simulink model "tg9"  (R2022a)
settings: Solver=ode15s  StartTime=0.0  StopTime=10  MaxStep=0.01  RelTol=1e-3
InitFcn:
  | mecha_param2
  | control_param0
values from neighbouring files (symbols this model uses):
  b0 = 0    [sim_IMMC.m]
  b1 = 1    [sim_IMMC.m]
  back0 = 0    [sim_IMMC.m]
  back1 = 0    [sim_IMMC.m]
  boff = 0    [sim_IMMC.m]
  bon = 0    [sim_IMMC.m]
  c = 0.05    [mecha_param2.m]
  c_jointstop = 0.3 / (pi/180)    (= 17.1887338539)    [mecha_param2.m]
  calctalus = sqrt((L_foot - (DJ1x_foot))^2 + (H_foot-r_cs)^2)    [mecha_param2.m]
  calctoes = sqrt((H_foot-r_cs)^2 + (DJ1x_foot)^2)    [mecha_param2.m]
  corrD = 0.001    [control_param0.m]
  DG_HAT = 0.35    [mecha_param2.m]
  DG_thigh = 0.28    [mecha_param2.m]
  DJ1x_foot = 0.16-r_cs    (= 0.135)    [mecha_param2.m]
  eref = 0.04    [mecha_param2.m]
  FmaxBFSH = 350    [mecha_param2.m]
  FmaxGAS = 1500    [mecha_param2.m]
  FmaxGLU = 1500    [mecha_param2.m]
  FmaxHAM = 3000    [mecha_param2.m]
  FmaxHFL = 2000    [mecha_param2.m]
  FmaxRF = 1200    [mecha_param2.m]
  FmaxSOL = 4000    [mecha_param2.m]
  FmaxTA = 800    [mecha_param2.m]
  FmaxVAS = 6000    [mecha_param2.m]
  g = 9.81    [mecha_param2.m]
  g0 = 0    [sim_IMMC.m]
  g1 = 0    [sim_IMMC.m]
  H_foot = 0.08    [mecha_param2.m]
  In_HAT = 3    [mecha_param2.m]
  In_shank = 0.05    [mecha_param2.m]
  In_thigh = 0.15    [mecha_param2.m]
  K = 5    [mecha_param2.m]
  knee_thigh = [0 0 -(L_thigh/2)]    [mecha_param2.m]
  Kpress = m_HAT * g / DeltaThRef    (= 104967)    [mecha_param2.m]
  L_foot = 0.2    [mecha_param2.m]
  L_HAT = 0.8    [mecha_param2.m]
  L_shank = 0.46    [mecha_param2.m]
  L_thigh = 0.46    [mecha_param2.m]
  LoHAM = table2array(mt('LoHAM', 1))    [control_param0.m]
  LoHFL = table2array(mt('LoHFL', 1))    [control_param0.m]
  longD = longD - corrD    (= 0.019)    [control_param0.m]
  loptBFSH = 0.12    [mecha_param2.m]
  loptGAS = 0.05    [mecha_param2.m]
  loptGLU = 0.11    [mecha_param2.m]
  loptHAM = 0.10    (= 0.1)    [mecha_param2.m]
  loptHFL = 0.11    [mecha_param2.m]
  loptRF = 0.08    [mecha_param2.m]
  loptSOL = 0.04    [mecha_param2.m]
  loptTA = 0.06    [mecha_param2.m]
  loptVAS = 0.08    [mecha_param2.m]
  LoTA = table2array(mt('LoTA', 1))    [control_param0.m]
  lslackBFSH = 0.10    (= 0.1)    [mecha_param2.m]
  lslackGAS = 0.40    (= 0.4)    [mecha_param2.m]
  lslackGLU = 0.13    [mecha_param2.m]
  lslackHAM = 0.31    [mecha_param2.m]
  lslackHFL = 0.10    (= 0.1)    [mecha_param2.m]
  lslackRF = 0.35    [mecha_param2.m]
  lslackSOL = 0.26    [mecha_param2.m]
  lslackTA = 0.24    [mecha_param2.m]
  lslackVAS = 0.23    [mecha_param2.m]
  m_HAT = 53.5    [mecha_param2.m]
  m_shank = 3.5    [mecha_param2.m]
  m_thigh = 8.5    [mecha_param2.m]
  midD = midD - corrD    (= 0.009)    [control_param0.m]
  N = 1.5    [mecha_param2.m]
  nonoff = 0    [control_param0.m]
  phi_a_low = (70) * (pi / 180)    (= 1.2217304764)    [mecha_param2.m]
  phi_a_up = (130) * (pi / 180)    (= 2.26892802759)    [mecha_param2.m]
  phi_dl = 180    [mecha_param2.m]
  phi_h = 230 * (pi / 180)    (= 4.01425727959)    [mecha_param2.m]
  phi_k = 175 * (pi / 180)    (= 3.05432619099)    [mecha_param2.m]
  phictoes = asind((DJ1y_foot-r_cs)/calctoes)    [mecha_param2.m]
  phimaxGASa = 100*pi/180    (= 1.74532925199)    [mecha_param2.m]
  phimaxGASk = 140*pi/180    (= 2.44346095279)    [mecha_param2.m]
  phimaxRFk = 165*pi/180    (= 2.87979326579)    [mecha_param2.m]
  phimaxSOL = 100*pi/180    (= 1.74532925199)    [mecha_param2.m]
  phimaxTA = 80*pi/180    (= 1.3962634016)    [mecha_param2.m]
  phimaxVAS = 165*pi/180    (= 2.87979326579)    [mecha_param2.m]
  phirefBFSH = 160*pi/180    (= 2.79252680319)    [mecha_param2.m]
  phirefGASa = 80*pi/180    (= 1.3962634016)    [mecha_param2.m]
  phirefGASk = 165*pi/180    (= 2.87979326579)    [mecha_param2.m]
  phirefGLU = 120*pi/180    (= 2.09439510239)    [mecha_param2.m]
  phirefHAMh = 150*pi/180    (= 2.61799387799)    [mecha_param2.m]
  phirefHAMk = 180*pi/180    (= 3.14159265359)    [mecha_param2.m]
  phirefHFL = 160*pi/180    (= 2.79252680319)    [mecha_param2.m]
  phirefRFh = 170*pi/180    (= 2.96705972839)    [mecha_param2.m]
  phirefRFk = 125*pi/180    (= 2.18166156499)    [mecha_param2.m]
  phirefSOL = 90*pi/180    (= 1.57079632679)    [mecha_param2.m]
  phirefTA = 110*pi/180    (= 1.91986217719)    [mecha_param2.m]
  phirefVAS = 120*pi/180    (= 2.09439510239)    [mecha_param2.m]
  phiScaleGASa = acos(rGASamin/rGASamax)/(phiminGASa-phimaxGASa)    [mecha_param2.m]
  phiScaleGASk = acos(rGASkmin/rGASkmax)/(phiminGASk-phimaxGASk)    [mecha_param2.m]
  phiScaleRFk = acos(rRFkmin/rRFkmax)/(phiminRFk-phimaxRFk)    [mecha_param2.m]
  phiScaleSOL = acos(rSOLmin/rSOLmax)/(phiminSOL-phimaxSOL)    [mecha_param2.m]
  phiScaleTA = acos(rTAmin/rTAmax)/(phiminTA-phimaxTA)    [mecha_param2.m]
  phiScaleVAS = acos(rVASmin/rVASmax)/(phiminVAS-phimaxVAS)    [mecha_param2.m]
  r1 = 0    [sim_IMMC.m]
  r_cs = 0.025    [mecha_param2.m]
  rBFSH = 0.04    [mecha_param2.m]
  rGASamax = 0.06    [mecha_param2.m]
  rGASkmax = 0.05    [mecha_param2.m]
  rGLU = 0.08    [mecha_param2.m]
  rHAMh = 0.08    [mecha_param2.m]
  rHAMk = 0.05    [mecha_param2.m]
  rHFL = 0.08    [mecha_param2.m]
  rhoBFSH = 0.7    [mecha_param2.m]
  rhoGASa = 0.7    [mecha_param2.m]
  rhoGASk = 0.7    [mecha_param2.m]
  rhoGLU = 0.5    [mecha_param2.m]
  rhoHAMh = 0.5    [mecha_param2.m]
  rhoHAMk = 0.5    [mecha_param2.m]
  rhoHFL = 0.5    [mecha_param2.m]
  rhoRFh = 0.3    [mecha_param2.m]
  rhoRFk = 0.5    [mecha_param2.m]
  rhoSOL = 0.5    [mecha_param2.m]
  rhoTA = 0.7    [mecha_param2.m]
  rhoVAS = 0.6    [mecha_param2.m]
  rRFh = 0.08    [mecha_param2.m]
  rRFkmax = 0.06    [mecha_param2.m]
  rSOLmax = 0.06    [mecha_param2.m]
  ... (+25 more)
undefined symbols (not defined in the file or in its folder): beta11, beta12, beta13, beta14, beta15, beta16, beta21, beta22, beta23, beta24, beta25, beta26, beta31, beta32, beta33, beta34, beta35, beta36, beta41, beta42, beta43, beta44, beta45, beta46, beta51, beta52, beta53, beta54, beta55, beta56, betab1, betab2, betab3, betab4, betab5, betab6, betap11, betap12, betap13, betap14, betap15, betap16, betap21, betap22, betap23, betap24, betap25, betap26, betap31, betap32, betap33, betap34, betap35, betap36, betap41, betap42, betap43, betap44, betap45, betap46 ... (+102)
libraries: sm_lib x89, simulink x72, nesl_utility x58, simulink_extras x18
(part 8 of 12)

== system tg9/Neural Control Layer/IMsRight ==
  right2left : Inport
  drivers : Inport  Port=2
  eta : Inport  Port=3
  triggers : Inport  Port=4
  Add{1..5,8} (6 alike) : Sum
  Add10 : Sum  Inputs=+++
  Add6 : Sum  Inputs=++++
  Add7 : Sum  Inputs=++++
  Add9 : Sum  Inputs=+++
  Bias{1..6} (6 alike) : Bias  Bias=-0.001  SaturateOnIntegerOverflow=off
  Cast To Double{,1..3} (4 alike) : DataTypeConversion  OutDataTypeStr=double  SaturateOnIntegerOverflow=off  RndMeth=Floor
  Demux : Demux  Outputs=6
  Demux1 : Demux  Outputs=5
  Demux2 : Demux  Outputs=5
  Demux3 : Demux  Outputs=3
  Demux4 : Demux  Outputs=5
  Demux5 : Demux  Outputs=8
  Hit Crossing{1..8} (8 alike) : HitCross  HitCrossingOffset=0.5  HitCrossingDirection=rising  ZeroCross=off
  IMx3 : Subsystem
      settings: PortSchema="{\"entries\":[{\"content\":{\"sides\":[{\"content\":{\"connectorIds\":[\"In1\"]},\"type\":\"ConnectorPlacement.EquallySpacedRectSide\",\"uuid\":\"605af916-6978-477d-a73f-0473cfddaa9b\"},{\"content\":{\"connectorIds\":[\"In4\",\"Out1\",\"Out2\"],\"side\":\"RIGHT\"},\"type\":\"ConnectorPlacement.EquallySpacedRectSide\",\"uuid\":\"ae4b258d-886c-42c2-bd45-f153a9ad36f8\"},{\"content\":{\"connectorIds\":[\"In2\"],\"side\":\"TOP\"},\"type\":\"ConnectorPlacement.EquallySpacedRectSide\",\"uuid\":\"4a03238d-2b6a-43dc-934f-97c6bc5fc8f2\"},{\"content\":{\"connectorIds\":[\"In3\"],\"side\":\"BOTTOM\"},\"type\":\"ConnectorPlacement.EquallySpacedRectSide\",\"uuid\":\"5d056236-5ce8-482a-98e4-2b75471ba733\"}]},\"type\":\"ConnectorPlacement.EquallySpacedConnector\",\"uuid\":\"c8afc41f-4e3a-4f48-b0c9-a380f8c80fc8\"}],\"packageUris\":[\"http://schema.mathworks.com/mf0/Connector/R2020b\"],\"version\":\"1.0\"}"
  Mux{,1..3,5} (5 alike) : Mux  Inputs=5
  Mux6 : Mux  Inputs=3
  Mux7 : Mux  Inputs=3
  S1 : Subsystem  TreatAsAtomicUnit=on
  S2 : Subsystem  TreatAsAtomicUnit=on
  S3 : Subsystem  TreatAsAtomicUnit=on
  S4 : Subsystem  TreatAsAtomicUnit=on
  S5 : Subsystem  TreatAsAtomicUnit=on
  Sx : Subsystem  TreatAsAtomicUnit=on
  Transport Delay{1..6} (6 alike) : TransportDelay  DelayTime=corrD
  Zero : Constant  Value=0  OutDataTypeStr=Inherit: Inherit via back propagation
  backwardpool : Subsystem
      settings: PortSchema="{\"entries\":[{\"content\":{\"sides\":[{\"content\":{\"connectorIds\":[\"In1\",\"In2\",\"In3\"]},\"type\":\"ConnectorPlacement.EquallySpacedRectSide\",\"uuid\":\"a61b6c6e-9e6f-45f2-b50f-9bcdc7a13346\"},{\"content\":{\"connectorIds\":[\"Out1\",\"Out2\"],\"side\":\"RIGHT\"},\"type\":\"ConnectorPlacement.EquallySpacedRectSide\",\"uuid\":\"1e8eaab5-7abe-40b4-aee2-b3f1e694b70c\"},{\"content\":{\"connectorIds\":[\"In4\",\"In5\"],\"side\":\"TOP\"},\"type\":\"ConnectorPlacement.EquallySpacedRectSide\",\"uuid\":\"0d5c3f76-1ab4-4f7c-806d-755b82fcb7e0\"},{\"content\":{\"connectorIds\":[\"Out3\",\"In6\"],\"side\":\"BOTTOM\"},\"type\":\"ConnectorPlacement.EquallySpacedRectSide\",\"uuid\":\"6e4a109d-fd90-45a6-b737-e259d18310f6\"}]},\"type\":\"ConnectorPlacement.EquallySpacedConnector\",\"uuid\":\"c9455465-31f2-4bd0-89ee-d0d51ed162fd\"}],\"packageUris\":[\"http://schema.mathworks.com/mf0/Connector/R2020b\"],\"version\":\"1.0\"}"
  etas2 : Constant  OutDataTypeStr=Inherit: Inherit via back propagation
  forwardpool : Subsystem
      settings: PortSchema="{\"entries\":[{\"content\":{\"sides\":[{\"content\":{\"connectorIds\":[\"In1\",\"In2\",\"In3\"]},\"type\":\"ConnectorPlacement.EquallySpacedRectSide\",\"uuid\":\"a61b6c6e-9e6f-45f2-b50f-9bcdc7a13346\"},{\"content\":{\"connectorIds\":[\"Out1\",\"Out2\"],\"side\":\"RIGHT\"},\"type\":\"ConnectorPlacement.EquallySpacedRectSide\",\"uuid\":\"1e8eaab5-7abe-40b4-aee2-b3f1e694b70c\"},{\"content\":{\"connectorIds\":[\"In4\",\"In5\"],\"side\":\"TOP\"},\"type\":\"ConnectorPlacement.EquallySpacedRectSide\",\"uuid\":\"0d5c3f76-1ab4-4f7c-806d-755b82fcb7e0\"},{\"content\":{\"connectorIds\":[\"Out3\",\"In6\",\"Out4\"],\"side\":\"BOTTOM\"},\"type\":\"ConnectorPlacement.EquallySpacedRectSide\",\"uuid\":\"6e4a109d-fd90-45a6-b737-e259d18310f6\"}]},\"type\":\"ConnectorPlacement.EquallySpacedConnector\",\"uuid\":\"c9455465-31f2-4bd0-89ee-d0d51ed162fd\"}],\"packageUris\":[\"http://schema.mathworks.com/mf0/Connector/R2020b\"],\"version\":\"1.0\"}"
  standingpool : Subsystem
      settings: PortSchema="{\"entries\":[{\"content\":{\"sides\":[{\"content\":{\"connectorIds\":[\"In1\",\"In2\",\"In3\"]},\"type\":\"ConnectorPlacement.EquallySpacedRectSide\",\"uuid\":\"b712be9c-ffb9-40b3-9573-f9951c2c9790\"},{\"content\":{\"connectorIds\":[\"Out1\",\"Out2\",\"Out3\"],\"side\":\"RIGHT\"},\"type\":\"ConnectorPlacement.EquallySpacedRectSide\",\"uuid\":\"8b219718-e783-4b0c-8b79-845ed528538f\"},{\"content\":{\"connectorIds\":[\"In4\"],\"side\":\"TOP\"},\"type\":\"ConnectorPlacement.EquallySpacedRectSide\",\"uuid\":\"e04791c1-32da-4b4e-9c5c-e19faa0d0170\"},{\"content\":{\"connectorIds\":[\"In5\",\"Out4\"],\"side\":\"BOTTOM\"},\"type\":\"ConnectorPlacement.EquallySpacedRectSide\",\"uuid\":\"996429ae-f4aa-4411-9589-2ace4ffd34b2\"}]},\"type\":\"ConnectorPlacement.EquallySpacedConnector\",\"uuid\":\"20796571-eb07-4761-9f65-93ae0d0a6d2c\"}],\"packageUris\":[\"http://schema.mathworks.com/mf0/Connector/R2020b\"],\"version\":\"1.0\"}"
  beta : Outport
  wires:
  backwardpool/2(beta) -> Add7/4
  forwardpool/4(beta) -> Add7/3
  Transport Delay5/1 -> Bias5/1, Mux5/1, Mux2/1
  standingpool/3(beta) -> Add7/2
  Add7/1 -> beta/1
  IMx3/2(beta) -> Add7/1
  Mux7/1 -> IMx3/2(drivers)
  Cast To Double3/1 -> Add6/1
  etas2/1 -> Mux6/2, Mux6/3
  Mux6/1 -> IMx3/4(eta)
  Mux5/1 -> backwardpool/3(ui)
  Transport Delay3/1 -> Bias1/1, Mux5/5, Mux2/5
  backwardpool/1(vartheta) -> Add9/3
  backwardpool/3(trigger_out) -> Add10/3
  Demux3/3 -> backwardpool/6(control)
  Demux/1 -> Mux6/1
  Hit Crossing8/1 -> Cast To Double3/1
  Demux5/1 -> Mux7/3, Hit Crossing8/1
  Cast To Double2/1 -> Add6/3
  Hit Crossing7/1 -> Cast To Double2/1
  Demux5/2 -> Mux7/2, Hit Crossing7/1
  eta/1 -> Demux/1
  Demux/6 -> Mux/5
  Demux/2 -> Mux/1
  Demux/5 -> Mux/4
  Demux/4 -> Mux/3
  Demux/3 -> Mux/2
  Sx/2(theta) -> IMx3/3(phase)
  Zero/1 -> Sx/1(phi)
  IMx3/1(vartheta) -> Sx/2(varthetau)
  Cast To Double1/1 -> Add6/2
  Hit Crossing6/1 -> Cast To Double1/1
  Demux5/3 -> Hit Crossing6/1, Mux7/1
  Transport Delay4/1 -> Bias6/1, IMx3/1(ui)
  Bias6/1 -> Add6/4
  Sx/1(u1) -> Transport Delay4/1
  Add6/1 -> Sx/Enable
  Add3/1 -> S1/Enable
  right2left/1 -> forwardpool/4(right2left), backwardpool/4(right2left)
  Mux/1 -> standingpool/3(eta), forwardpool/1(eta), backwardpool/1(eta)
  Demux5/5 -> Hit Crossing1/1
  triggers/1 -> Demux5/1
  Mux1/1 -> forwardpool/2(phase), standingpool/1(phase), backwardpool/2(phase)
  S1/2(theta) -> Mux1/1
  S2/2(theta) -> Mux1/2
  S3/2(theta) -> Mux1/3
  Demux1/1 -> S1/1(phi)
  Demux1/2 -> S2/2(phi)
  Demux1/3 -> S3/2(phi)
  S1/1(u1) -> Transport Delay5/1
  S2/1(u2) -> Transport Delay6/1
  S3/1(u3) -> Transport Delay1/1
  S4/1(u3) -> Transport Delay2/1
  Demux1/4 -> S4/2(phi)
  S4/2(theta) -> Mux1/4
  S5/2(theta) -> Mux1/5
  Demux1/5 -> S5/2(phi)
  S5/1(u3) -> Transport Delay3/1
  Demux5/4 -> Hit Crossing2/1
  Mux2/1 -> forwardpool/3(ui), standingpool/2(ui)
  standingpool/1(vartheta) -> Add9/1
  forwardpool/2(vartheta) -> Add9/2
  Demux2/1 -> S1/2(varthetau)
  Add9/1 -> Demux2/1
  Add8/1 -> Demux1/1
  Demux2/2 -> S2/1(varthetau)
  Demux2/3 -> S3/1(varthetau)
  Demux2/4 -> S4/1(varthetau)
  Demux2/5 -> S5/1(varthetau)
  drivers/1 -> Demux3/1
  Bias2/1 -> Add4/2
  forwardpool/1(phi) -> Add8/2
  standingpool/2(phi) -> Add8/1
  Demux3/2 -> forwardpool/6(control)
  Demux3/1 -> standingpool/5(control)
  Bias1/1 -> Add5/2
  Bias3/1 -> Add2/2
  Bias4/1 -> Add1/2
  Bias5/1 -> Add3/2
  Add1/1 -> S2/Enable
  Add2/1 -> S3/Enable
  Add4/1 -> S4/Enable
  Add5/1 -> S5/Enable
  Demux5/6 -> Hit Crossing3/1
  Demux5/7 -> Hit Crossing4/1
  Demux5/8 -> Hit Crossing5/1
  Hit Crossing5/1 -> Mux3/5
  Hit Crossing4/1 -> Mux3/4
  Hit Crossing3/1 -> Mux3/3
  Hit Crossing1/1 -> Mux3/2
  Hit Crossing2/1 -> Mux3/1
  Mux3/1 -> Cast To Double/1
  forwardpool/3(trigger_out) -> Add10/2
  Add10/1 -> Demux4/1
  Demux4/1 -> Add3/1
  Demux4/2 -> Add1/1
  Demux4/3 -> Add2/1
  Demux4/4 -> Add4/1
  Demux4/5 -> Add5/1
  standingpool/4(trigger_out) -> Add10/1
  Cast To Double/1 -> standingpool/4(triggers), backwardpool/5(triggers), forwardpool/5(triggers)
  Transport Delay6/1 -> Bias4/1, Mux5/2, Mux2/2
  Transport Delay1/1 -> Bias3/1, Mux5/3, Mux2/3
  Transport Delay2/1 -> Bias2/1, Mux5/4, Mux2/4

== system tg9/Neural Control Layer/Subsystem1 ==
  In1 : Inport
  m : Inport  Port=2
  In2 : Inport  Port=3
  Constant : Constant  Value=mim2
  Constant1 : Constant  Value=mi
  Demux : Demux  Outputs=2
  Mux : Mux  Inputs=2
  Product : Product
  Product1 : Product
  Saturation : Saturate  UpperLimit=inf  LowerLimit=0  ZeroCross=off
  Sum : Sum  Inputs=++|
  Out1 : Outport
  Out2 : Outport  Port=2
  wires:
  Sum/1 -> Product1/1
  m/1 -> Product/2
  Product/1 -> Sum/1
  Constant1/1 -> Sum/2
  Constant/1 -> Product/1
  Mux/1 -> Product1/2
  Product1/1 -> Saturation/1
  Saturation/1 -> Demux/1
  Demux/1 -> Out1/1
  Demux/2 -> Out2/1
  In2/1 -> Mux/2
  In1/1 -> Mux/1

== system tg9/Neural Control Layer/Subsystem2 ==
  In1 : Inport
  m : Inport  Port=2
  In2 : Inport  Port=3
  Constant : Constant  Value=mim3
  Constant1 : Constant  Value=mi
  Demux : Demux  Outputs=2
  Mux : Mux  Inputs=2
  Product : Product
  Product1 : Product
  Saturation : Saturate  UpperLimit=inf  LowerLimit=0  ZeroCross=off
  Sum : Sum  Inputs=++|
  Out1 : Outport
  Out2 : Outport  Port=2
  wires:
  In1/1 -> Mux/1
  In2/1 -> Mux/2
  Demux/2 -> Out2/1
  Demux/1 -> Out1/1
  Saturation/1 -> Demux/1
  Product1/1 -> Saturation/1
  Mux/1 -> Product1/2
  Constant/1 -> Product/1
  Constant1/1 -> Sum/2
  Product/1 -> Sum/1
  m/1 -> Product/2
  Sum/1 -> Product1/1

== system tg9/Neural Control Layer/Subsystem3 ==
  In1 : Inport
  m : Inport  Port=2
  In2 : Inport  Port=3
  Constant : Constant  Value=mim1
  Constant1 : Constant  Value=mi
  Demux : Demux  Outputs=2
  Mux : Mux  Inputs=2
  Product : Product
  Product1 : Product
  Saturation : Saturate  UpperLimit=inf  LowerLimit=0  ZeroCross=off
  Sum : Sum  Inputs=++|
  Out1 : Outport
  Out2 : Outport  Port=2
  wires:
  In1/1 -> Mux/1
  In2/1 -> Mux/2
  Demux/2 -> Out2/1
  Demux/1 -> Out1/1
  Saturation/1 -> Demux/1
  Product1/1 -> Saturation/1
  Mux/1 -> Product1/2
  Constant/1 -> Product/1
  Constant1/1 -> Sum/2
  Product/1 -> Sum/1
  m/1 -> Product/2
  Sum/1 -> Product1/1

== system tg9/Neural Control Layer/Subsystem4 ==
  In1 : Inport
  m : Inport  Port=2
  In2 : Inport  Port=3
  Constant : Constant  Value=mim2
  Constant1 : Constant  Value=mi
  Demux : Demux  Outputs=2
  Mux : Mux  Inputs=2
  Product : Product
  Product1 : Product
  Saturation : Saturate  UpperLimit=inf  LowerLimit=0  ZeroCross=off
  Sum : Sum  Inputs=++|
  Out1 : Outport
  Out2 : Outport  Port=2
  wires:
  Sum/1 -> Product1/1
  m/1 -> Product/2
  Product/1 -> Sum/1
  Constant1/1 -> Sum/2
  Constant/1 -> Product/1
  Mux/1 -> Product1/2
  Product1/1 -> Saturation/1
  Saturation/1 -> Demux/1
  Demux/1 -> Out1/1
  Demux/2 -> Out2/1
  In2/1 -> Mux/2
  In1/1 -> Mux/1

== system tg9/Neural Control Layer/Subsystem5 ==
  In1 : Inport
  m : Inport  Port=2
  In2 : Inport  Port=3
  Constant : Constant  Value=mim3
  Constant1 : Constant  Value=mi
  Demux : Demux  Outputs=2
  Mux : Mux  Inputs=2
  Product : Product
  Product1 : Product
  Saturation : Saturate  UpperLimit=inf  LowerLimit=0  ZeroCross=off
  Sum : Sum  Inputs=++|
  Out1 : Outport
  Out2 : Outport  Port=2
  wires:
  In1/1 -> Mux/1
  In2/1 -> Mux/2
  Demux/2 -> Out2/1
  Demux/1 -> Out1/1
  Saturation/1 -> Demux/1
  Product1/1 -> Saturation/1
  Mux/1 -> Product1/2
  Constant/1 -> Product/1
  Constant1/1 -> Sum/2
  Product/1 -> Sum/1
  m/1 -> Product/2
  Sum/1 -> Product1/1

== system tg9/Neural Control Layer/Subsystem6 ==
  In1 : Inport
  m : Inport  Port=2
  In2 : Inport  Port=3
  Constant : Constant  Value=mim1
  Constant1 : Constant  Value=mi
  Demux : Demux  Outputs=2
  Mux : Mux  Inputs=2
  Product : Product
  Product1 : Product
  Saturation : Saturate  UpperLimit=inf  LowerLimit=0  ZeroCross=off
  Sum : Sum  Inputs=++|
  Out1 : Outport
  Out2 : Outport  Port=2
  wires:
  In1/1 -> Mux/1
  In2/1 -> Mux/2
  Demux/2 -> Out2/1
  Demux/1 -> Out1/1
  Saturation/1 -> Demux/1
  Product1/1 -> Saturation/1
  Mux/1 -> Product1/2
  Constant/1 -> Product/1
  Constant1/1 -> Sum/2
  Product/1 -> Sum/1
  m/1 -> Product/2
  Sum/1 -> Product1/1

== system tg9/Neural Control Layer/noisy ==
  In1 : Inport
  Add9 : Sum
  Divide8 : Product  Inputs=**
  Gain4 : Gain  Gain=nonoff
  Random Number3 : RandomNumber  Variance=var_noise  Seed=4  SampleTime=1/80
  Out1 : Outport
  wires:
  In1/1 -> Divide8/1, Add9/1
  Random Number3/1 -> Gain4/1
  Gain4/1 -> Divide8/2
  Divide8/1 -> Add9/2
  Add9/1 -> Out1/1

== system tg9/Neural Control Layer/noisy1 ==
  In1 : Inport
  Add9 : Sum
  Divide8 : Product  Inputs=**
  Gain4 : Gain  Gain=nonoff
  Random Number3 : RandomNumber  Variance=var_noise  Seed=3  SampleTime=1/80
  Out1 : Outport
  wires:
  Add9/1 -> Out1/1
  Divide8/1 -> Add9/2
  Gain4/1 -> Divide8/2
  Random Number3/1 -> Gain4/1
  In1/1 -> Add9/1, Divide8/1

== system tg9/Neural Control Layer/noisy10 ==
  In1 : Inport
  Add9 : Sum
  Divide8 : Product  Inputs=**
  Gain4 : Gain  Gain=nonoff
  Random Number3 : RandomNumber  Variance=var_noise  Seed=1  SampleTime=1/80
  Out1 : Outport
  wires:
  Add9/1 -> Out1/1
  Divide8/1 -> Add9/2
  Gain4/1 -> Divide8/2
  Random Number3/1 -> Gain4/1
  In1/1 -> Add9/1, Divide8/1

== system tg9/Neural Control Layer/noisy11 ==
  In1 : Inport
  Add9 : Sum
  Divide8 : Product  Inputs=**
  Gain4 : Gain  Gain=nonoff
  Random Number3 : RandomNumber  Variance=var_noise  Seed=6  SampleTime=1/80
  Out1 : Outport
  wires:
  In1/1 -> Divide8/1, Add9/1
  Random Number3/1 -> Gain4/1
  Gain4/1 -> Divide8/2
  Divide8/1 -> Add9/2
  Add9/1 -> Out1/1

== system tg9/Neural Control Layer/noisy2 ==
  In1 : Inport
  Add9 : Sum
  Divide8 : Product  Inputs=**
  Gain4 : Gain  Gain=nonoff
  Random Number3 : RandomNumber  Variance=var_noise  Seed=2  SampleTime=1/80
  Out1 : Outport
  wires:
  In1/1 -> Divide8/1, Add9/1
  Random Number3/1 -> Gain4/1
  Gain4/1 -> Divide8/2
  Divide8/1 -> Add9/2
  Add9/1 -> Out1/1

== system tg9/Neural Control Layer/noisy3 ==
  In1 : Inport
  Add9 : Sum
  Divide8 : Product  Inputs=**
  Gain4 : Gain  Gain=nonoff
  Random Number3 : RandomNumber  Variance=var_noise  Seed=5  SampleTime=1/80
  Out1 : Outport
  wires:
  Add9/1 -> Out1/1
  Divide8/1 -> Add9/2
  Gain4/1 -> Divide8/2
  Random Number3/1 -> Gain4/1
  In1/1 -> Add9/1, Divide8/1

== system tg9/Neural Control Layer/noisy4 ==
  In1 : Inport
  Add9 : Sum
  Divide8 : Product  Inputs=**
  Gain4 : Gain  Gain=nonoff
  Random Number3 : RandomNumber  Variance=var_noise  Seed=6  SampleTime=1/80
  Out1 : Outport
  wires:
  In1/1 -> Divide8/1, Add9/1
  Random Number3/1 -> Gain4/1
  Gain4/1 -> Divide8/2
  Divide8/1 -> Add9/2
  Add9/1 -> Out1/1

== system tg9/Neural Control Layer/noisy5 ==
  In1 : Inport
  Add9 : Sum
  Divide8 : Product  Inputs=**
  Gain4 : Gain  Gain=nonoff
  Random Number3 : RandomNumber  Variance=var_noise  Seed=1  SampleTime=1/80
  Out1 : Outport
  wires:
  In1/1 -> Divide8/1, Add9/1
  Random Number3/1 -> Gain4/1
  Gain4/1 -> Divide8/2
  Divide8/1 -> Add9/2
  Add9/1 -> Out1/1

== system tg9/Neural Control Layer/noisy6 ==
  In1 : Inport
  Add9 : Sum
  Divide8 : Product  Inputs=**
  Gain4 : Gain  Gain=nonoff
  Random Number3 : RandomNumber  Variance=var_noise  Seed=7  SampleTime=1/80
  Out1 : Outport
  wires:
  In1/1 -> Divide8/1, Add9/1
  Random Number3/1 -> Gain4/1
  Gain4/1 -> Divide8/2
  Divide8/1 -> Add9/2
  Add9/1 -> Out1/1

== system tg9/Neural Control Layer/noisy7 ==
  In1 : Inport
  Add9 : Sum
  Divide8 : Product  Inputs=**
  Gain4 : Gain  Gain=nonoff
  Random Number3 : RandomNumber  Variance=var_noise  Seed=5  SampleTime=1/80
  Out1 : Outport
  wires:
  In1/1 -> Divide8/1, Add9/1
  Random Number3/1 -> Gain4/1
  Gain4/1 -> Divide8/2
  Divide8/1 -> Add9/2
  Add9/1 -> Out1/1

== system tg9/Neural Control Layer/noisy8 ==
  In1 : Inport
  Add9 : Sum
  Divide8 : Product  Inputs=**
  Gain4 : Gain  Gain=nonoff
  Random Number3 : RandomNumber  Variance=var_noise  Seed=3  SampleTime=1/80
  Out1 : Outport
  wires:
  In1/1 -> Divide8/1, Add9/1
  Random Number3/1 -> Gain4/1
  Gain4/1 -> Divide8/2
  Divide8/1 -> Add9/2
  Add9/1 -> Out1/1

== system tg9/Neural Control Layer/noisy9 ==
  In1 : Inport
  Add9 : Sum
  Divide8 : Product  Inputs=**
  Gain4 : Gain  Gain=nonoff
  Random Number3 : RandomNumber  Variance=var_noise  Seed=2  SampleTime=1/80
  Out1 : Outport
  wires:
  Add9/1 -> Out1/1
  Divide8/1 -> Add9/2
  Gain4/1 -> Divide8/2
  Random Number3/1 -> Gain4/1
  In1/1 -> Add9/1, Divide8/1

== system tg9/Body Mechanics Layer/Left Leg/Left Thigh ==
  note: Left Thigh Sensor Sheet
  note: I do not know where this formula comes from, but I do suppose that it keeps the thigh not altered
  Gain : Gain  Gain=Kpress
  Gain1 : Gain  Gain=1/vmaxpress
  Gain5 : Gain  Gain=-1
  L Low Thigh trans : sm_lib/Frames and Transforms/Rigid Transform  TranslationMethod=Cartesian  TranslationStandardOffset=0  TranslationLengthUnit=m  TranslationStandardAxis=+Z  TranslationCartesianOffset=[0 0 -L_thigh/2] * (ThPos)  TranslationROffset=0  TranslationROffsetUnits=m  TranslationZOffset=0  TranslationZOffsetUnits=m  TranslationThetaOffset=0  TranslationThetaOffsetUnits=deg  RotationMethod=None  RotationAngleUnits=deg  RotationStandardAxis=+Z  RotationAngle=0.0  RotationArbitraryAxis=[0 0 1]  FollAlignAxisA=+X  BaseAlignAxisA=+Y  FollAlignAxisB=+Y  BaseAlignAxisB=+Z  RotationSequenceAxes=FollowerAxes  RotationSequence=XYX  RotationSequenceAngles=[0 0 0]  RotationSequenceAnglesUnits=deg  RotationMatrix=[1 0 0; 0 1 0; 0 0 1]
  L Prism Joint trans : sm_lib/Frames and Transforms/Rigid Transform  TranslationMethod=Cartesian  TranslationStandardOffset=0  TranslationLengthUnit=m  TranslationStandardAxis=+Z  TranslationCartesianOffset=[0 0 -L_thigh/2] * (1-ThPos)  TranslationROffset=0  TranslationROffsetUnits=m  TranslationZOffset=0  TranslationZOffsetUnits=m  TranslationThetaOffset=0  TranslationThetaOffsetUnits=deg  RotationMethod=None  RotationAngleUnits=deg  RotationStandardAxis=+Z  RotationAngle=0.0  RotationArbitraryAxis=[0 0 1]  FollAlignAxisA=+X  BaseAlignAxisA=+Y  FollAlignAxisB=+Y  BaseAlignAxisB=+Z  RotationSequenceAxes=FollowerAxes  RotationSequence=XYX  RotationSequenceAngles=[0 0 0]  RotationSequenceAnglesUnits=deg  RotationMatrix=[1 0 0; 0 1 0; 0 0 1]
  L Prismatic Joint : sm_lib/Joints/Prismatic Joint  JointMode=Normal  SenseConstraintForce=off  SenseConstraintForceX=off  SenseConstraintForceY=off  SenseConstraintForceZ=off  SenseConstraintTorque=off  SenseConstraintTorqueX=off  SenseConstraintTorqueY=off  SenseConstraintTorqueZ=off  SenseTotalForce=off  SenseTotalForceX=off  SenseTotalForceY=off  SenseTotalForceZ=off  SenseTotalTorque=off  SenseTotalTorqueX=off  SenseTotalTorqueY=off  SenseTotalTorqueZ=off  CompositeWrenchDir=FollowerOnBase  CompositeWrenchFrame=BaseFrame  EquilibriumPosition=0  EquilibriumPositionUnits=m  SpringStiffness=0  SpringStiffnessUnits=N/m  DampingCoefficient=0  DampingCoefficientUnits=N/(m/s)  TorqueActuationMode=InputTorque  MotionActuationMode=ComputedMotion  SensePosition=on  SenseVelocity=on  SenseAcceleration=off  SenseTorqueForce=off  SenseLowerLimitTorqueForce=off  SenseUpperLimitTorqueForce=off  LowerLimitSpecify=off  LowerLimitBound=-1  LowerLimitBoundUnits=m  LowerLimitStiffness=1e6  LowerLimitStiffnessUnits=N/m  LowerLimitDamping=1e3  LowerLimitDampingUnits=N/(m/s)  LowerLimitTransitionRegionWidth=1e-4  LowerLimitTransitionRegionWidthUnits=m  UpperLimitSpecify=off  UpperLimitBound=1  UpperLimitBoundUnits=m  UpperLimitStiffness=1e6  UpperLimitStiffnessUnits=N/m  UpperLimitDamping=1e3  UpperLimitDampingUnits=N/(m/s)  UpperLimitTransitionRegionWidth=1e-4  UpperLimitTransitionRegionWidthUnits=m  PositionTargetSpecify=off  PositionTargetPriority=High  PositionTargetValue=0  PositionTargetValueUnits=m  VelocityTargetSpecify=off  VelocityTargetPriority=High  VelocityTargetValue=0  VelocityTargetValueUnits=m/s
  Left High Thigh : sm_lib/Body Elements/Cylindrical Solid  GraphicAmbientColor=[0.15 0.15 0.15 1.0]  BasedOnType=Density  CenterOfMass=[0 0 -((L_thigh/2)-DG_thigh)] * (1-ThPos)  CenterOfMassUnits=m  GraphicDiffuseColor=bcolor  CylinderLength=L_thigh * (1-ThPos)  CylinderLengthUnits=m  CylinderRadius=r_thigh  CylinderRadiusUnits=m  Density=1000  DensityUnits=kg/m^3  DoExposeReferenceFrame=on  GraphicEmissiveColor=[0.0 0.0 0.0 1.0]  ExportEntireGeometry=off  SerializedFrames=<Frames/>  MarkerShape=Sphere  MarkerSize=10  GraphicType=FromGeometry  InertiaType=Custom  Mass=m_thigh * (1-ThPos)  MassUnits=kg  MomentsOfInertia=[1 0 0]*In_thigh * (1-ThPos)  MomentsOfInertiaUnits=kg*m^2  GraphicOpacity=1.0  ProductsOfInertia=[0 0 0]  ProductsOfInertiaUnits=kg*m^2  GraphicShininess=75  GraphicSpecularColor=[0.5 0.5 0.5 1.0]  GraphicVisPropType=SimpleVisualProperties
  Left Low Thigh : sm_lib/Body Elements/Cylindrical Solid  GraphicAmbientColor=[0.15 0.15 0.15 1.0]  BasedOnType=Density  CenterOfMass=[0 0 -((L_thigh/2)-DG_thigh)] * (ThPos)  CenterOfMassUnits=m  GraphicDiffuseColor=[0.5 0.5 0.5]  CylinderLength=L_thigh * ThPos  CylinderLengthUnits=m  CylinderRadius=r_thigh  CylinderRadiusUnits=m  Density=1000  DensityUnits=kg/m^3  DoExposeReferenceFrame=on  GraphicEmissiveColor=[0.0 0.0 0.0 1.0]  ExportEntireGeometry=off  SerializedFrames=<Frames/>  MarkerShape=Sphere  MarkerSize=10  GraphicType=FromGeometry  InertiaType=Custom  Mass=m_thigh * (ThPos)  MassUnits=kg  MomentsOfInertia=[1 0 0]*In_thigh * (ThPos)  MomentsOfInertiaUnits=kg*m^2  GraphicOpacity=1.0  ProductsOfInertia=[0 0 0]  ProductsOfInertiaUnits=kg*m^2  GraphicShininess=75  GraphicSpecularColor=[0.5 0.5 0.5 1.0]  GraphicVisPropType=SimpleVisualProperties
  Mux : Mux  Inputs=2
  PS-Simulink Converter : nesl_utility/PS-Simulink Converter  PhysicalDomain=network_engine_domain  SubClassName=ps_output  LeftPortType=input  RightPortType=output  PseudoPeriodic=off  Frequencies=[]  VectorFormat=1-D array  Unit=inherit  AffineConversion=off
      settings: SourceProductBaseCode=SS,PW,VE
  PS-Simulink Converter1 : nesl_utility/PS-Simulink Converter  PhysicalDomain=network_engine_domain  SubClassName=ps_output  LeftPortType=input  RightPortType=output  PseudoPeriodic=off  Frequencies=[]  VectorFormat=1-D array  Unit=inherit  AffineConversion=off
      settings: SourceProductBaseCode=SS,PW,VE
  Pressure Sheet Reaction Force : Fcn  Expr=-u(1) * (1+sgn(u(1))*u(2))
  Scope : Scope
  Simulink-PS Converter : nesl_utility/Simulink-PS Converter  PhysicalDomain=network_engine_domain  SubClassName=ps_input  LeftPortType=input  RightPortType=output  PseudoPeriodic=off  Frequencies=[]  NoiseDistribution=none  NoiseParameters=[]  Unit=1  AffineConversion=off  FilteringAndDerivatives=provide  SimscapeFilterOrder=1  InputFilterTimeConstant=0.001  UdotUserProvided=0
      settings: SourceProductBaseCode=SS,PW,VE
  from L hip : PMIOPort  Side=Left
  to L knee : PMIOPort  Port=2  Side=Right
  dx : Outport
  wires:
  Mux/1 -> Pressure Sheet Reaction Force/1
  Gain/1 -> Mux/1
  Gain1/1 -> Mux/2
  PS-Simulink Converter/1 -> Gain/1, Gain5/1
  PS-Simulink Converter1/1 -> Gain1/1, Scope/1
  Pressure Sheet Reaction Force/1 -> Simulink-PS Converter/1
  Gain5/1 -> dx/1
  connections:
  from L hip/RConn1 -- Left High Thigh/RConn1 -- L Prism Joint trans/LConn1
  Left Low Thigh/RConn1 -- to L knee/RConn1 -- L Low Thigh trans/RConn1
  Simulink-PS Converter/RConn1 -- L Prismatic Joint/LConn2
  PS-Simulink Converter/LConn1 -- L Prismatic Joint/RConn2
  PS-Simulink Converter1/LConn1 -- L Prismatic Joint/RConn3
  L Low Thigh trans/LConn1 -- L Prismatic Joint/LConn1
  L Prismatic Joint/RConn1 -- L Prism Joint trans/RConn1

== system tg9/Body Mechanics Layer/Right Leg/Right Thigh ==
  note: Right Thigh Sensor Sheet
  note: I do not know where this formula comes from, but I do suppose that it keeps the thigh not altered
  Gain : Gain  Gain=Kpress
  Gain1 : Gain  Gain=1/vmaxpress
  Gain5 : Gain  Gain=-1
  Mux : Mux  Inputs=2
  PS-Simulink Converter : nesl_utility/PS-Simulink Converter  PhysicalDomain=network_engine_domain  SubClassName=ps_output  LeftPortType=input  RightPortType=output  PseudoPeriodic=off  Frequencies=[]  VectorFormat=1-D array  Unit=inherit  AffineConversion=off
      settings: SourceProductBaseCode=SS,PW,VE
  PS-Simulink Converter1 : nesl_utility/PS-Simulink Converter  PhysicalDomain=network_engine_domain  SubClassName=ps_output  LeftPortType=input  RightPortType=output  PseudoPeriodic=off  Frequencies=[]  VectorFormat=1-D array  Unit=inherit  AffineConversion=off
      settings: SourceProductBaseCode=SS,PW,VE
  Pressure Sheet Reaction Force : Fcn  Expr=-u(1) * (1+sgn(u(1))*u(2))
  R Low Thigh trans : sm_lib/Frames and Transforms/Rigid Transform  TranslationMethod=Cartesian  TranslationStandardOffset=0  TranslationLengthUnit=m  TranslationStandardAxis=+Z  TranslationCartesianOffset=[0 0 -L_thigh/2] * (ThPos)  TranslationROffset=0  TranslationROffsetUnits=m  TranslationZOffset=0  TranslationZOffsetUnits=m  TranslationThetaOffset=0  TranslationThetaOffsetUnits=deg  RotationMethod=None  RotationAngleUnits=deg  RotationStandardAxis=+Z  RotationAngle=0.0  RotationArbitraryAxis=[0 0 1]  FollAlignAxisA=+X  BaseAlignAxisA=+Y  FollAlignAxisB=+Y  BaseAlignAxisB=+Z  RotationSequenceAxes=FollowerAxes  RotationSequence=XYX  RotationSequenceAngles=[0 0 0]  RotationSequenceAnglesUnits=deg  RotationMatrix=[1 0 0; 0 1 0; 0 0 1]
  R Prism Joint trans : sm_lib/Frames and Transforms/Rigid Transform  TranslationMethod=Cartesian  TranslationStandardOffset=0  TranslationLengthUnit=m  TranslationStandardAxis=+Z  TranslationCartesianOffset=[0 0 -L_thigh/2] * (1-ThPos)  TranslationROffset=0  TranslationROffsetUnits=m  TranslationZOffset=0  TranslationZOffsetUnits=m  TranslationThetaOffset=0  TranslationThetaOffsetUnits=deg  RotationMethod=None  RotationAngleUnits=deg  RotationStandardAxis=+Z  RotationAngle=0.0  RotationArbitraryAxis=[0 0 1]  FollAlignAxisA=+X  BaseAlignAxisA=+Y  FollAlignAxisB=+Y  BaseAlignAxisB=+Z  RotationSequenceAxes=FollowerAxes  RotationSequence=XYX  RotationSequenceAngles=[0 0 0]  RotationSequenceAnglesUnits=deg  RotationMatrix=[1 0 0; 0 1 0; 0 0 1]
  R Prismatic Joint : sm_lib/Joints/Prismatic Joint  JointMode=Normal  SenseConstraintForce=off  SenseConstraintForceX=off  SenseConstraintForceY=off  SenseConstraintForceZ=off  SenseConstraintTorque=off  SenseConstraintTorqueX=off  SenseConstraintTorqueY=off  SenseConstraintTorqueZ=off  SenseTotalForce=off  SenseTotalForceX=off  SenseTotalForceY=off  SenseTotalForceZ=off  SenseTotalTorque=off  SenseTotalTorqueX=off  SenseTotalTorqueY=off  SenseTotalTorqueZ=off  CompositeWrenchDir=FollowerOnBase  CompositeWrenchFrame=BaseFrame  EquilibriumPosition=0  EquilibriumPositionUnits=m  SpringStiffness=0  SpringStiffnessUnits=N/m  DampingCoefficient=0  DampingCoefficientUnits=N/(m/s)  TorqueActuationMode=InputTorque  MotionActuationMode=ComputedMotion  SensePosition=on  SenseVelocity=on  SenseAcceleration=off  SenseTorqueForce=off  SenseLowerLimitTorqueForce=off  SenseUpperLimitTorqueForce=off  LowerLimitSpecify=off  LowerLimitBound=-1  LowerLimitBoundUnits=m  LowerLimitStiffness=1e6  LowerLimitStiffnessUnits=N/m  LowerLimitDamping=1e3  LowerLimitDampingUnits=N/(m/s)  LowerLimitTransitionRegionWidth=1e-4  LowerLimitTransitionRegionWidthUnits=m  UpperLimitSpecify=off  UpperLimitBound=1  UpperLimitBoundUnits=m  UpperLimitStiffness=1e6  UpperLimitStiffnessUnits=N/m  UpperLimitDamping=1e3  UpperLimitDampingUnits=N/(m/s)  UpperLimitTransitionRegionWidth=1e-4  UpperLimitTransitionRegionWidthUnits=m  PositionTargetSpecify=off  PositionTargetPriority=High  PositionTargetValue=0  PositionTargetValueUnits=m  VelocityTargetSpecify=off  VelocityTargetPriority=High  VelocityTargetValue=0  VelocityTargetValueUnits=m/s
  Right High Thigh : sm_lib/Body Elements/Cylindrical Solid  GraphicAmbientColor=[0.15 0.15 0.15 1.0]  BasedOnType=Density  CenterOfMass=[0 0 -((L_thigh/2)-DG_thigh)] * (1-ThPos)  CenterOfMassUnits=m  GraphicDiffuseColor=bcolor  CylinderLength=L_thigh * (1-ThPos)  CylinderLengthUnits=m  CylinderRadius=r_thigh  CylinderRadiusUnits=m  Density=1000  DensityUnits=kg/m^3  DoExposeReferenceFrame=on  GraphicEmissiveColor=[0.0 0.0 0.0 1.0]  ExportEntireGeometry=off  SerializedFrames=<Frames/>  MarkerShape=Sphere  MarkerSize=10  GraphicType=FromGeometry  InertiaType=Custom  Mass=m_thigh * (1-ThPos)  MassUnits=kg  MomentsOfInertia=[1 0 0]*In_thigh * (1-ThPos)  MomentsOfInertiaUnits=kg*m^2  GraphicOpacity=1.0  ProductsOfInertia=[0 0 0]  ProductsOfInertiaUnits=kg*m^2  GraphicShininess=75  GraphicSpecularColor=[0.5 0.5 0.5 1.0]  GraphicVisPropType=SimpleVisualProperties
  Right Low Thigh : sm_lib/Body Elements/Cylindrical Solid  GraphicAmbientColor=[0.15 0.15 0.15 1.0]  BasedOnType=Density  CenterOfMass=[0 0 -((L_thigh/2)-DG_thigh)] * (ThPos)  CenterOfMassUnits=m  GraphicDiffuseColor=[0.5 0.5 0.5]  CylinderLength=L_thigh * ThPos  CylinderLengthUnits=m  CylinderRadius=r_thigh  CylinderRadiusUnits=m  Density=1000  DensityUnits=kg/m^3  DoExposeReferenceFrame=on  GraphicEmissiveColor=[0.0 0.0 0.0 1.0]  ExportEntireGeometry=off  SerializedFrames=<Frames/>  MarkerShape=Sphere  MarkerSize=10  GraphicType=FromGeometry  InertiaType=Custom  Mass=m_thigh * (ThPos)  MassUnits=kg  MomentsOfInertia=[1 0 0]*In_thigh * (ThPos)  MomentsOfInertiaUnits=kg*m^2  GraphicOpacity=1.0  ProductsOfInertia=[0 0 0]  ProductsOfInertiaUnits=kg*m^2  GraphicShininess=75  GraphicSpecularColor=[0.5 0.5 0.5 1.0]  GraphicVisPropType=SimpleVisualProperties
  Scope : Scope
  Simulink-PS Converter : nesl_utility/Simulink-PS Converter  PhysicalDomain=network_engine_domain  SubClassName=ps_input  LeftPortType=input  RightPortType=output  PseudoPeriodic=off  Frequencies=[]  NoiseDistribution=none  NoiseParameters=[]  Unit=1  AffineConversion=off  FilteringAndDerivatives=provide  SimscapeFilterOrder=1  InputFilterTimeConstant=0.001  UdotUserProvided=0
      settings: SourceProductBaseCode=SS,PW,VE
  from R hip : PMIOPort  Side=Left
  to R knee : PMIOPort  Port=2  Side=Right
  dx : Outport
  wires:
  Mux/1 -> Pressure Sheet Reaction Force/1
  Gain/1 -> Mux/1
  Gain1/1 -> Mux/2
  Pressure Sheet Reaction Force/1 -> Scope/1, Simulink-PS Converter/1
  PS-Simulink Converter/1 -> Gain/1, Gain5/1
  PS-Simulink Converter1/1 -> Gain1/1
  Gain5/1 -> dx/1
  connections:
  from R hip/RConn1 -- R Prism Joint trans/LConn1 -- Right High Thigh/RConn1
  Right Low Thigh/RConn1 -- to R knee/RConn1 -- R Low Thigh trans/RConn1
  Simulink-PS Converter/RConn1 -- R Prismatic Joint/LConn2
  PS-Simulink Converter/LConn1 -- R Prismatic Joint/RConn2
  PS-Simulink Converter1/LConn1 -- R Prismatic Joint/RConn3
  R Low Thigh trans/LConn1 -- R Prismatic Joint/LConn1
  R Prismatic Joint/RConn1 -- R Prism Joint trans/RConn1

== system tg9/Muscle Actuation Layer/L BFSH/BE force-length relation ==
  note: fbe, compression force-length relationship
  note: ((lce+w-1)/(w/2))^2
  note: lce[lopt]-(1-w)
  note: if lce<1-w
  note: reference compression
  lce [lopt] : Inport
  Constant : Constant  Value=w/2
  Constant1 : Constant  Value=1-w
  Math Function : Math  Operator=square
  Mux : Mux  Inputs=2
  Sum : Sum  Inputs=|+-
  excentric branch1 : Fcn  Expr=u(2)*(u(1)<0)
  relative strain : Product  Inputs=*/
  fbe [Fmax] : Outport
  wires:
  Math Function/1 -> Mux/2
  Constant/1 -> relative strain/2
  lce [lopt]/1 -> Sum/1
  Sum/1 -> relative strain/1, Mux/1
  Constant1/1 -> Sum/2
  relative strain/1 -> Math Function/1
  Mux/1 -> excentric branch1/1
  excentric branch1/1 -> fbe [Fmax]/1

== system tg9/Muscle Actuation Layer/L BFSH/CE force-length relation ==
  note: (|lce-1|/w)^3
  note: |lce-1|/w
  note: |lce-1|
  note: lce-1
  note: fce, force-length relationship
  lce [lopt] : Inport
  Abs : Abs  SaturateOnIntegerOverflow=off
  Constant : Constant
  Constant1 : Constant  Value=w
  Constant2 : Constant  Value=3
  Exp : Math
  Exp1 : Math  Operator=pow  SignedPower=on
  Gain : Gain  Gain=log(c)
  Sum : Sum  Inputs=|+-
  normalized position : Product  Inputs=*/
  fce [Fmax] : Outport
  wires:
  Exp/1 -> fce [Fmax]/1
  Gain/1 -> Exp/1
  Exp1/1 -> Gain/1
  Constant2/1 -> Exp1/2
  normalized position/1 -> Exp1/1
  Abs/1 -> normalized position/1
  Sum/1 -> Abs/1
  Constant1/1 -> normalized position/2
  Constant/1 -> Sum/2
  lce [lopt]/1 -> Sum/1

== system tg9/Muscle Actuation Layer/L BFSH/CE inverse force-velocity relation ==
  note: fv-1
  note: 1+K*fv
  note: K*fv
  note: CE, inverse force-velocity relationship
  note: u(1) * (u(2)<=1)
  Fv[Fmax] : Inport
  Constant{,1,3..4} (4 alike) : Constant
  Constant2 : Constant  Value=N
  Constant5 : Constant  Value=N
  Divide2 : Product  Inputs=/*
  Divide3 : Product  Inputs=*/
  Gain : Gain  Gain=K
  Gain2 : Gain  Gain=7.56*K
  Gain3 : Gain  Gain=1e-2
  Mux : Mux  Inputs=3
  Mux1 : Mux  Inputs=2
  Mux2 : Mux  Inputs=3
  Product : Product  Inputs=*/
  Sum : Sum  Inputs=|+-
  Sum1 : Sum  Inputs=++|
  Sum2 : Sum  Inputs=+|+
  Sum3 : Sum  Inputs=+|+
  Sum4 : Sum  Inputs=-+|
  Sum5 : Sum  Inputs=|-+
  Sum6 : Sum  Inputs=|++
  Sum7 : Sum  Inputs=+-|
  Sum8 : Sum  Inputs=|++
  excentric branch1 : Fcn  Expr=u(2) * (u(1)>1)*(u(1)<=u(3))
  excentric branch2 : Fcn  Expr=u(1) * (u(2)<=1)
  excentric branch3 : Fcn  Expr=u(3) * (u(2)>u(1))
  v[vmax] : Outport
  wires:
  Fv[Fmax]/1 -> Sum4/2, Sum/1, Gain/1, Mux1/2, Mux2/1, Mux/2
  Sum2/1 -> Sum3/2
  excentric branch3/1 -> Sum2/2
  excentric branch1/1 -> Sum2/1
  Mux/1 -> excentric branch3/1
  Mux2/1 -> excentric branch1/1
  Constant5/1 -> Mux2/3, Mux/1
  Divide3/1 -> Mux2/2
  Sum8/1 -> Mux/3
  Constant4/1 -> Sum8/2
  Gain3/1 -> Sum8/1
  Gain2/1 -> Sum7/2
  Sum7/1 -> Divide3/2
  Divide2/1 -> Sum6/1, Gain2/1
  Constant/1 -> Sum6/2, Sum7/1
  Sum6/1 -> Divide3/1
  Sum4/1 -> Divide2/2, Gain3/1
  Sum5/1 -> Divide2/1
  Constant3/1 -> Sum5/1
  Constant2/1 -> Sum4/1, Sum5/2
  Sum3/1 -> v[vmax]/1
  excentric branch2/1 -> Sum3/1
  Mux1/1 -> excentric branch2/1
  Product/1 -> Mux1/1
  Sum1/1 -> Product/2
  Gain/1 -> Sum1/2
  Constant1/1 -> Sum1/1, Sum/2
  Sum/1 -> Product/1

== system tg9/Muscle Actuation Layer/L BFSH/PE force-length relation ==
  note: fpe, force-length relationship
  note: ((lce-1)/w)^2
  note: lce-1
  note: if lse > 1
  note: tendon reference strain, relative to lslack
  lce [lopt] : Inport
  Constant : Constant  Value=w
  Constant1 : Constant
  Math Function : Math  Operator=square
  Mux : Mux  Inputs=2
  Sum : Sum  Inputs=|+-
  excentric branch1 : Fcn  Expr=u(2) * (u(1)>1)
  relative strain : Product  Inputs=*/
  fpe [Fmax] : Outport
  wires:
  Math Function/1 -> Mux/2
  Constant/1 -> relative strain/2
  lce [lopt]/1 -> Sum/1, Mux/1
  Sum/1 -> relative strain/1
  Constant1/1 -> Sum/2
  relative strain/1 -> Math Function/1
  Mux/1 -> excentric branch1/1
  excentric branch1/1 -> fpe [Fmax]/1

== system tg9/Muscle Actuation Layer/L BFSH/SE force-length relation ==
  note: e>0 or lse>1
  note: (e/eref)^2
  note: e = (lse-lslack)/lslack;
      | e = lse[lslack]-1
  note: tendon reference strain, relative to lslack
  note: fse, elastic force-length relationship
  lse [lslack] : Inport
  Constant : Constant  Value=eref
  Constant1 : Constant
  Math Function : Math  Operator=square
  Mux : Mux  Inputs=2
  Sum : Sum  Inputs=|+-
  excentric branch1 : Fcn  Expr=u(2)*(u(1)>1)
  relative strain : Product  Inputs=*/
  fse [Fmax] : Outport
  wires:
  excentric branch1/1 -> fse [Fmax]/1
  Mux/1 -> excentric branch1/1
  Math Function/1 -> Mux/2
  relative strain/1 -> Math Function/1
  Constant/1 -> relative strain/2
  Constant1/1 -> Sum/2
  Sum/1 -> relative strain/1
  lse [lslack]/1 -> Sum/1, Mux/1

== system tg9/Muscle Actuation Layer/L GAS/BE force-length relation ==
  note: reference compression
  note: if lce<1-w
  note: lce[lopt]-(1-w)
  note: ((lce+w-1)/(w/2))^2
  note: fbe, compression force-length relationship
  lce [lopt] : Inport
  Constant : Constant  Value=w/2
  Constant1 : Constant  Value=1-w
  Math Function : Math  Operator=square
  Mux : Mux  Inputs=2
  Sum : Sum  Inputs=|+-
  excentric branch1 : Fcn  Expr=u(2)*(u(1)<0)
  relative strain : Product  Inputs=*/
  fbe [Fmax] : Outport
  wires:
  excentric branch1/1 -> fbe [Fmax]/1
  Mux/1 -> excentric branch1/1
  relative strain/1 -> Math Function/1
  Constant1/1 -> Sum/2
  Sum/1 -> Mux/1, relative strain/1
  lce [lopt]/1 -> Sum/1
  Constant/1 -> relative strain/2
  Math Function/1 -> Mux/2

== system tg9/Muscle Actuation Layer/L GAS/CE force-length relation ==
  note: fce, force-length relationship
  note: lce-1
  note: |lce-1|
  note: |lce-1|/w
  note: (|lce-1|/w)^3
  lce [lopt] : Inport
  Abs : Abs  SaturateOnIntegerOverflow=off
  Constant : Constant
  Constant1 : Constant  Value=w
  Constant2 : Constant  Value=3
  Exp : Math
  Exp1 : Math  Operator=pow  SignedPower=on
  Gain : Gain  Gain=log(c)
  Sum : Sum  Inputs=|+-
  normalized position : Product  Inputs=*/
  fce [Fmax] : Outport
  wires:
  lce [lopt]/1 -> Sum/1
  Constant/1 -> Sum/2
  Constant1/1 -> normalized position/2
  Sum/1 -> Abs/1
  Abs/1 -> normalized position/1
  normalized position/1 -> Exp1/1
  Constant2/1 -> Exp1/2
  Exp1/1 -> Gain/1
  Gain/1 -> Exp/1
  Exp/1 -> fce [Fmax]/1

== system tg9/Muscle Actuation Layer/L GAS/CE inverse force-velocity relation ==
  note: u(1) * (u(2)<=1)
  note: CE, inverse force-velocity relationship
  note: K*fv
  note: 1+K*fv
  note: fv-1
  Fv[Fmax] : Inport
  Constant{,1,3..4} (4 alike) : Constant
  Constant2 : Constant  Value=N
  Constant5 : Constant  Value=N
  Divide2 : Product  Inputs=/*
  Divide3 : Product  Inputs=*/
  Gain : Gain  Gain=K
  Gain2 : Gain  Gain=7.56*K
  Gain3 : Gain  Gain=1e-2
  Mux : Mux  Inputs=3
  Mux1 : Mux  Inputs=2
  Mux2 : Mux  Inputs=3
  Product : Product  Inputs=*/
  Sum : Sum  Inputs=|+-
  Sum1 : Sum  Inputs=++|
  Sum2 : Sum  Inputs=+|+
  Sum3 : Sum  Inputs=+|+
  Sum4 : Sum  Inputs=-+|
  Sum5 : Sum  Inputs=|-+
  Sum6 : Sum  Inputs=|++
  Sum7 : Sum  Inputs=+-|
  Sum8 : Sum  Inputs=|++
  excentric branch1 : Fcn  Expr=u(2) * (u(1)>1)*(u(1)<=u(3))
  excentric branch2 : Fcn  Expr=u(1) * (u(2)<=1)
  excentric branch3 : Fcn  Expr=u(3) * (u(2)>u(1))
  v[vmax] : Outport
  wires:
  Sum/1 -> Product/1
  Constant1/1 -> Sum/2, Sum1/1
  Gain/1 -> Sum1/2
  Sum1/1 -> Product/2
  Product/1 -> Mux1/1
  Mux1/1 -> excentric branch2/1
  excentric branch2/1 -> Sum3/1
  Sum3/1 -> v[vmax]/1
  Constant2/1 -> Sum5/2, Sum4/1
  Constant3/1 -> Sum5/1
  Sum5/1 -> Divide2/1
  Sum4/1 -> Gain3/1, Divide2/2
  Sum6/1 -> Divide3/1
  Constant/1 -> Sum7/1, Sum6/2
  Divide2/1 -> Gain2/1, Sum6/1
  Sum7/1 -> Divide3/2
  Gain2/1 -> Sum7/2
  Gain3/1 -> Sum8/1
  Constant4/1 -> Sum8/2
  Sum8/1 -> Mux/3
  Divide3/1 -> Mux2/2
  Constant5/1 -> Mux/1, Mux2/3
  Mux2/1 -> excentric branch1/1
  Mux/1 -> excentric branch3/1
  excentric branch1/1 -> Sum2/1
  excentric branch3/1 -> Sum2/2
  Sum2/1 -> Sum3/2
  Fv[Fmax]/1 -> Mux/2, Mux2/1, Mux1/2, Gain/1, Sum/1, Sum4/2

== system tg9/Muscle Actuation Layer/L GAS/PE force-length relation ==
  note: tendon reference strain, relative to lslack
  note: if lse > 1
  note: lce-1
  note: ((lce-1)/w)^2
  note: fpe, force-length relationship
  lce [lopt] : Inport
  Constant : Constant  Value=w
  Constant1 : Constant
  Math Function : Math  Operator=square
  Mux : Mux  Inputs=2
  Sum : Sum  Inputs=|+-
  excentric branch1 : Fcn  Expr=u(2) * (u(1)>1)
  relative strain : Product  Inputs=*/
  fpe [Fmax] : Outport
  wires:
  excentric branch1/1 -> fpe [Fmax]/1
  Mux/1 -> excentric branch1/1
  relative strain/1 -> Math Function/1
  Constant1/1 -> Sum/2
  Sum/1 -> relative strain/1
  lce [lopt]/1 -> Mux/1, Sum/1
  Constant/1 -> relative strain/2
  Math Function/1 -> Mux/2

== system tg9/Muscle Actuation Layer/L GAS/SE force-length relation ==
  note: fse, elastic force-length relationship
  note: tendon reference strain, relative to lslack
  note: e = (lse-lslack)/lslack;
      | e = lse[lslack]-1
  note: (e/eref)^2
  note: e>0 or lse>1
  lse [lslack] : Inport
  Constant : Constant  Value=eref
  Constant1 : Constant
  Math Function : Math  Operator=square
  Mux : Mux  Inputs=2
  Sum : Sum  Inputs=|+-
  excentric branch1 : Fcn  Expr=u(2)*(u(1)>1)
  relative strain : Product  Inputs=*/
  fse [Fmax] : Outport
  wires:
  lse [lslack]/1 -> Mux/1, Sum/1
  Sum/1 -> relative strain/1
  Constant1/1 -> Sum/2
  Constant/1 -> relative strain/2
  relative strain/1 -> Math Function/1
  Math Function/1 -> Mux/2
  Mux/1 -> excentric branch1/1
  excentric branch1/1 -> fse [Fmax]/1

== system tg9/Muscle Actuation Layer/L GLU/BE force-length relation ==
  note: reference compression
  note: if lce<1-w
  note: lce[lopt]-(1-w)
  note: ((lce+w-1)/(w/2))^2
  note: fbe, compression force-length relationship
  lce [lopt] : Inport
  Constant : Constant  Value=w/2
  Constant1 : Constant  Value=1-w
  Math Function : Math  Operator=square
  Mux : Mux  Inputs=2
  Sum : Sum  Inputs=|+-
  excentric branch1 : Fcn  Expr=u(2)*(u(1)<0)
  relative strain : Product  Inputs=*/
  fbe [Fmax] : Outport
  wires:
  excentric branch1/1 -> fbe [Fmax]/1
  Mux/1 -> excentric branch1/1
  relative strain/1 -> Math Function/1
  Constant1/1 -> Sum/2
  Sum/1 -> Mux/1, relative strain/1
  lce [lopt]/1 -> Sum/1
  Constant/1 -> relative strain/2
  Math Function/1 -> Mux/2

== system tg9/Muscle Actuation Layer/L GLU/CE force-length relation ==
  note: fce, force-length relationship
  note: lce-1
  note: |lce-1|
  note: |lce-1|/w
  note: (|lce-1|/w)^3
  lce [lopt] : Inport
  Abs : Abs  SaturateOnIntegerOverflow=off
  Constant : Constant
  Constant1 : Constant  Value=w
  Constant2 : Constant  Value=3
  Exp : Math
  Exp1 : Math  Operator=pow  SignedPower=on
  Gain : Gain  Gain=log(c)
  Sum : Sum  Inputs=|+-
  normalized position : Product  Inputs=*/
  fce [Fmax] : Outport
  wires:
  lce [lopt]/1 -> Sum/1
  Constant/1 -> Sum/2
  Constant1/1 -> normalized position/2
  Sum/1 -> Abs/1
  Abs/1 -> normalized position/1
  normalized position/1 -> Exp1/1
  Constant2/1 -> Exp1/2
  Exp1/1 -> Gain/1
  Gain/1 -> Exp/1
  Exp/1 -> fce [Fmax]/1
